simulink model "Lab11_CompFilter_13b"  (R2013b)
settings: Solver=FixedStepDiscrete  SolverMode=SingleTasking  StartTime=0.0  StopTime=inf  FixedStep=sim_step_size  RelTol=1e-3
PreLoadFcn:
  | %
  | C2D = 0.5
  | sim_step_size = 0.03
  | 
  | % Default parameters
  | Vs = 4.5;
  | Gyro_Bias = -247;
libraries: simulink x1
settings Model: SimulationMode=external  ExtModeTrigDuration=2  Creator=nding  LastModifiedBy=nding
settings OptimizationCC: OptimizeModelRefInitCode=on  LifeSpan=1
settings DebuggingCC: SolverPrmCheckMsg=none
settings HardwareCC: ProdBitPerInt=16  ProdBitPerPointer=8  ProdIntDivRoundTo=Zero  ProdEndianess=LittleEndian  ProdWordSize=8  ProdHWDeviceType=Atmel->AVR
settings RTWCC: SystemTargetFile=realtime.tlc  GenerateMakefile=off  TemplateMakefile=realtime.tmf  Description=Run on Target Hardware  RTWVerbose=off  ProcessScript=realtime_make_rtw_hook
settings STFCustomTargetCC: TargetLibSuffix=.a  GenerateSampleERTMain=on  ERTCustomFileBanners=on  SupportNonInlinedSFcns=off  SupportVariableSizeSignals=on  MATLABClassNameForMDSCustomization=Simulink.SoftwareTarget.ERTCustomization  GRTInterface=off  SystemTargetFile=realtime.tlc
settings ERTTargetCC: CodeReplacementLibrary=ANSI_C  GenerateSampleERTMain=on  ParMdlRefBuildCompliant=off  CompOptLevelCompliant=off  ConcurrentExecutionCompliant=off  CombineOutputUpdateFcns=off  ERTFirstTimeCompliant=off  SupportContinuousTime=on  SupportVariableSizeSignals=on  ModelStepFunctionPrototypeControlCompliant=off  CPPClassGenCompliant=off  ExtMode=on  ExtModeTransport=3  ExtModeMexArgs=0 11 115200 30  InlinedParameterPlacement=NonHierarchical  ERTSrcFileBannerTemplate=realtime_code_template.cgt  ERTHdrFileBannerTemplate=realtime_code_template.cgt  ERTDataSrcFileTemplate=realtime_code_template.cgt  ERTDataHdrFileTemplate=realtime_code_template.cgt  ERTCustomFileTemplate=realtime_file_process.tlc

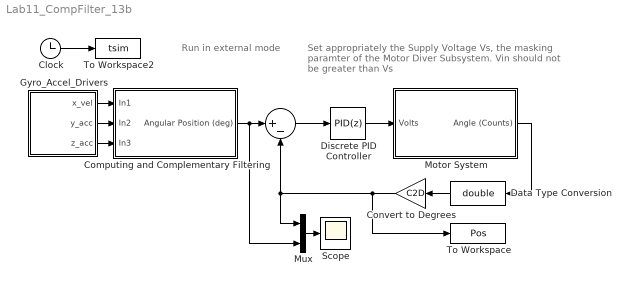
== system Lab11_CompFilter_13b ==
  note: Set appropriately the Supply  Voltage Vs, the masking paramter
      | of the Motor Diver Subsystem. Vin should not  be greater than Vs
  note: Run in external mode
  " " : Sum  Inputs=|+-
  Clock : Clock
  Computing and Complementary Filtering : Subsystem
  Convert to Degrees : Gain  Gain=C2D
  Data Type Conversion : DataTypeConversion  OutDataTypeStr=double
  Discrete PID Controller : simulink/Continuous/PID Controller  Controller=PID  TimeDomain=Discrete-time  SampleTime=sim_step_size  IntegratorMethod=Forward Euler  FilterMethod=Forward Euler  Form=Parallel  P=0.1  I=0  D=0  N=100  InitialConditionSource=internal  InitialConditionForIntegrator=0  InitialConditionForFilter=0  ExternalReset=none  LimitOutput=off  UpperSaturationLimit=inf  LowerSaturationLimit=-inf  LinearizeAsGain=off  AntiWindupMode=none  Kb=1  TrackingMode=off  Kt=1  PParamMin=[]  PParamMax=[]  IParamMin=[]  IParamMax=[]  DParamMin=[]  DParamMax=[]  NParamMin=[]  NParamMax=[]  KbParamMin=[]  KbParamMax=[]  KtParamMin=[]  KtParamMax=[]  POutMin=[]  POutMax=[]  IOutMin=[]  IOutMax=[]  DOutMin=[]  DOutMax=[]  NOutMin=[]  NOutMax=[]  KbOutMin=[]  KbOutMax=[]  KtOutMin=[]  KtOutMax=[]  IntegratorOutMin=[]  IntegratorOutMax=[]  FilterOutMin=[]  FilterOutMax=[]  SumOutMin=[]  SumOutMax=[]  SumI1OutMin=[]  SumI1OutMax=[]  SumI2OutMin=[]  SumI2OutMax=[]  SumI3OutMin=[]  SumI3OutMax=[]  SumDOutMin=[]  SumDOutMax=[]  SaturationOutMin=[]  SaturationOutMax=[]  IntegratorContinuousStateAttributes=''  IntegratorStateMustResolveToSignalObject=off  IntegratorRTWStateStorageClass=Auto  FilterContinuousStateAttributes=''  FilterStateMustResolveToSignalObject=off  FilterRTWStateStorageClass=Auto
  Gyro_Accel_Drivers : Subsystem
  Motor System : Subsystem
  Mux : Mux  Inputs=2
  Scope : Scope
      settings: YMin=0  YMax=100
  To Workspace : ToWorkspace  VariableName=Pos  SampleTime=-1
  To Workspace2 : ToWorkspace  VariableName=tsim  SampleTime=sim_step_size
  wires:
  Motor System/1(Angle (Counts)) -> Data Type Conversion/1
  Discrete PID Controller/1 -> Motor System/1(Volts)
  Clock/1 -> To Workspace2/1
  " "/1 -> Discrete PID Controller/1
  Computing and Complementary Filtering/1(Angular Position (deg)) -> " "/1, Mux/2
  Data Type Conversion/1 -> Convert to Degrees/1
  Convert to Degrees/1 -> To Workspace/1, Mux/1, " "/2
  Mux/1 -> Scope/1
  Gyro_Accel_Drivers/1(x_vel) -> Computing and Complementary Filtering/1(In1)
  Gyro_Accel_Drivers/2(y_acc) -> Computing and Complementary Filtering/2(In2)
  Gyro_Accel_Drivers/3(z_acc) -> Computing and Complementary Filtering/3(In3)

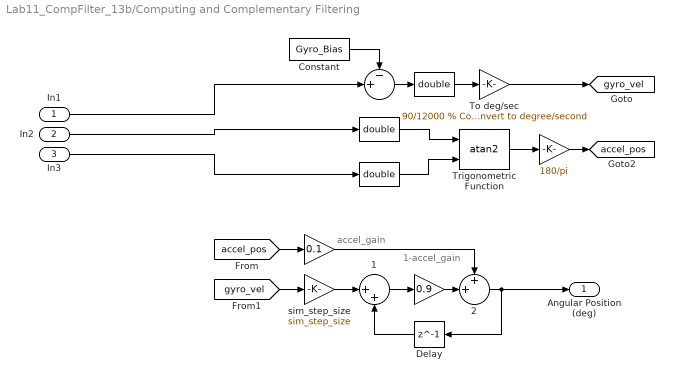
== system Lab11_CompFilter_13b/Computing and Complementary Filtering ==
  note: 1-accel_gain
  note: accel_gain
  In1 : Inport
  In2 : Inport  Port=2
  In3 : Inport  Port=3
  " " : Sum  Inputs=-+|
  "  " : DataTypeConversion  OutDataTypeStr=double
  "   " : DataTypeConversion  OutDataTypeStr=double
  "    " : Gain  Gain=0.1
  "     " : DataTypeConversion  OutDataTypeStr=double
  "      " : Gain  Gain=180/pi
  "          " : Gain  Gain=0.9
  "    sim_step_size" : Gain  Gain=sim_step_size
  " 1" : Sum  Inputs=|++
  " 2" : Sum  Inputs=++|
  Constant : Constant  Value=Gyro_Bias
  Delay : Delay  DelayLength=1
  To deg/sec : Gain  Gain=90/12000 % Convert to degree/second
  Trigonometric Function : Trigonometry  Operator=atan2
  Angular Position (deg) : Outport
  tag scope: accel_pos=global, gyro_vel=global
  wires:
  In2/1 -> "   "/1
  In3/1 -> "     "/1
  In1/1 -> " "/2
  Trigonometric Function/1 -> "      "/1
  [gyro_vel] -> "    sim_step_size"/1
  "   "/1 -> Trigonometric Function/1
  "      "/1 -> [accel_pos]
  "     "/1 -> Trigonometric Function/2
  "  "/1 -> To deg/sec/1
  "    "/1 -> " 2"/1
  Constant/1 -> " "/1
  "          "/1 -> " 2"/2
  To deg/sec/1 -> [gyro_vel]
  " 2"/1 -> Angular Position (deg)/1, Delay/1
  "    sim_step_size"/1 -> " 1"/1
  Delay/1 -> " 1"/2
  " "/1 -> "  "/1
  " 1"/1 -> "          "/1
  [accel_pos] -> "    "/1

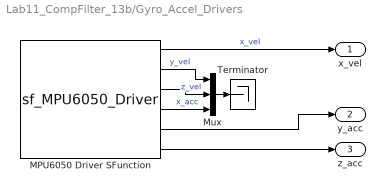
== system Lab11_CompFilter_13b/Gyro_Accel_Drivers ==
  MPU6050 Driver SFunction : S-Function  InitFcn=try, set_param(gcb,'FunctionName','sf_MPU6050_Driver'), end  FunctionName=sf_MPU6050_Driver  SFunctionModules=sf_MPU6050_Driver_wrapper  EnableBusSupport=off  mask(S-Function Builder){}
      mask help: Simulink:masks:SFunctionBuilder_MD
      mask init:
      | val = [[.9  0.75 0.75 1 1 .9 .9 1]',[1 1 0.75 0.75 .9 .9 1 .9]'];try , sys = get_param(gcb,'SfunBuilderFcnName');if isempty(sys), sys = get_param(gcb,'FunctionName'); end,catch, sys = get_param(gcb,'FunctionName'); end
      settings: CopyFcn=set_param(gcbh,'LinkStatus','none')  PreSaveFcn=try, set_param(gcb,'FunctionName','sf_MPU6050_Driver'), end  OpenFcn=sfunctionwizard(gcbh)
      mask Display: plot(val(:,1),val(:,2)),disp(sys), port_label('output',1,'x_vel'), port_label('output',2,'y_vel'), port_label('output',3,'z_vel'), port_label('output',4,'x_acc'), port_label('output',5,'y_acc'), port_label('output',6,'z_acc')
  Mux : Mux  Inputs=3
  Terminator : Terminator
  x_vel : Outport
  y_acc : Outport  Port=2
  z_acc : Outport  Port=3
  wires:
  Mux/1 -> Terminator/1
  MPU6050 Driver SFunction/4 -> Mux/3  "x_acc"
  MPU6050 Driver SFunction/5 -> y_acc/1
  MPU6050 Driver SFunction/6 -> z_acc/1
  MPU6050 Driver SFunction/1 -> x_vel/1  "x_vel"
  MPU6050 Driver SFunction/2 -> Mux/1  "y_vel"
  MPU6050 Driver SFunction/3 -> Mux/2  "z_vel"

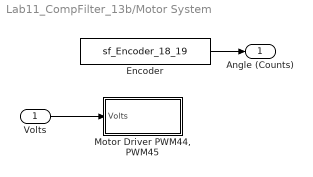
== system Lab11_CompFilter_13b/Motor System ==
  Volts : Inport
  Encoder : S-Function  InitFcn=try, set_param(gcb,'FunctionName','sf_Encoder_18_19'), end  FunctionName=sf_Encoder_18_19  Parameters=uint8(0),uint8(18),uint8(19)  SFunctionModules=sf_Encoder_18_19_wrapper  EnableBusSupport=off  mask(S-Function Builder){}
      mask init: same as Lab11_CompFilter_13b/Gyro_Accel_Drivers/MPU6050 Driver SFunction
      settings: CopyFcn=set_param(gcbh,'LinkStatus','none')  PreSaveFcn=try, set_param(gcb,'FunctionName','sf_Encoder_18_19'), end  OpenFcn=sfunctionwizard(gcbh)
      mask Display: plot(val(:,1),val(:,2)),disp(sys), port_label('output',1,'pos')
  "Motor Driver PWM44, PWM45" : Subsystem  mask{Vs=Vs, Delta=0}
      mask prompts: Vs "Supply Voltage Vs: USB 4.5v; Battery 9v"; Delta "PWM Offset Delta: 0-255"
      mask init:
      | Vusb=4.5;
      | Vbat=9.0;
      mask DialogControl T Prompt: Specify Motor Supply Voltage and PWM Offset
  Angle (Counts) : Outport
  wires:
  Encoder/1 -> Angle (Counts)/1
  Volts/1 -> "Motor Driver PWM44, PWM45"/1(Volts)

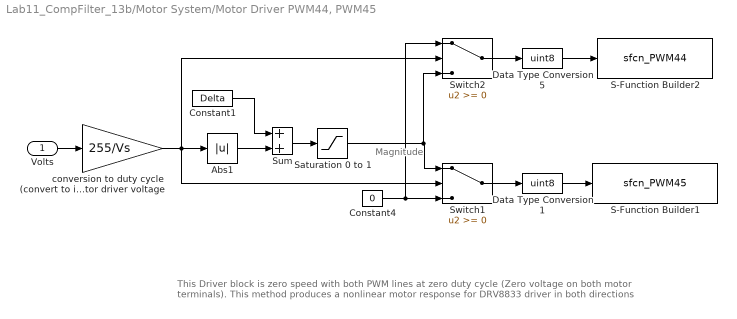
== system Lab11_CompFilter_13b/Motor System/Motor Driver PWM44, PWM45 ==
  note: Magnitude
  note: This Driver block is zero speed with both PWM lines at zero duty cycle  (Zero voltage on both motor terminals).
      | This method produces a nonlinear motor response for DRV8833 driver in both directions
  Volts : Inport
  Abs1 : Abs
  Constant1 : Constant  Value=Delta
  Constant4 : Constant  Value=0
  Data Type Conversion1 : DataTypeConversion  OutDataTypeStr=uint8
  Data Type Conversion5 : DataTypeConversion  OutDataTypeStr=uint8
  S-Function Builder1 : S-Function  InitFcn=try, set_param(gcb,'FunctionName','sfcn_PWM45'), end  FunctionName=sfcn_PWM45  Parameters=uint8(45)  SFunctionModules=sfcn_PWM45_wrapper  EnableBusSupport=off  mask(S-Function Builder){}
      mask init: same as Lab11_CompFilter_13b/Gyro_Accel_Drivers/MPU6050 Driver SFunction
      settings: CopyFcn=set_param(gcbh,'LinkStatus','none')  PreSaveFcn=try, set_param(gcb,'FunctionName','sfcn_PWM45'), end  OpenFcn=sfunctionwizard(gcbh)
      mask Display: plot(val(:,1),val(:,2)),disp(sys), port_label('input',1,'in')
  S-Function Builder2 : S-Function  InitFcn=try, set_param(gcb,'FunctionName','sfcn_PWM44'), end  FunctionName=sfcn_PWM44  Parameters=uint8(44)  SFunctionModules=sfcn_PWM44_wrapper  EnableBusSupport=off  mask(S-Function Builder){}
      mask init: same as Lab11_CompFilter_13b/Gyro_Accel_Drivers/MPU6050 Driver SFunction
      settings: CopyFcn=set_param(gcbh,'LinkStatus','none')  PreSaveFcn=try, set_param(gcb,'FunctionName','sfcn_PWM44'), end  OpenFcn=sfunctionwizard(gcbh)
      mask Display: plot(val(:,1),val(:,2)),disp(sys), port_label('input',1,'in')
  Saturation 0 to 1 : Saturate  UpperLimit=255  LowerLimit=0
  Sum : Sum
  Switch1 : Switch
  Switch2 : Switch
  conversion to duty cycle (convert to int) denominator is motor driver voltage : Gain  Gain=255/Vs  OutDataTypeStr=int16
  wires:
  Constant1/1 -> Sum/1
  Sum/1 -> Saturation 0 to 1/1
  Abs1/1 -> Sum/2
  Data Type Conversion1/1 -> S-Function Builder1/1
  Data Type Conversion5/1 -> S-Function Builder2/1
  Switch1/1 -> Data Type Conversion1/1
  Switch2/1 -> Data Type Conversion5/1
  Saturation 0 to 1/1 -> Switch1/1, Switch2/3
  Constant4/1 -> Switch1/3, Switch2/1
  conversion to duty cycle (convert to int) denominator is motor driver voltage/1 -> Switch2/2, Abs1/1, Switch1/2
  Volts/1 -> conversion to duty cycle (convert to int) denominator is motor driver voltage/1
